simulink model "SistemaP4"  (R2023a)
settings: Solver=VariableStepAuto  StartTime=0.0  StopTime=10.0  MaxStep=1e-3  RelTol=1e-3
libraries: fl_lib x7, nesl_utility x3, slpidlib x1
settings Model: Creator=gabri  LastModifiedBy=gabri
settings DataIOCC: SaveOutput=off  SignalLogging=off  DSMLogging=off  ReturnWorkspaceOutputs=off  TimeSaveName=t
settings DebuggingCC: AlgebraicLoopMsg=none  ArtificialAlgebraicLoopMsg=none  MaxConsecutiveZCsMsg=none  ModelReferenceExtraNoncontSigs=none  OperatingPointInterfaceChecksumMismatchMsg=none

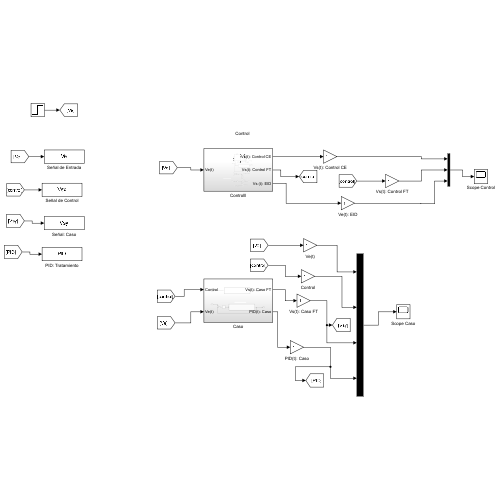
[thumbnail: Simulink's stored preview of the top-level diagram]
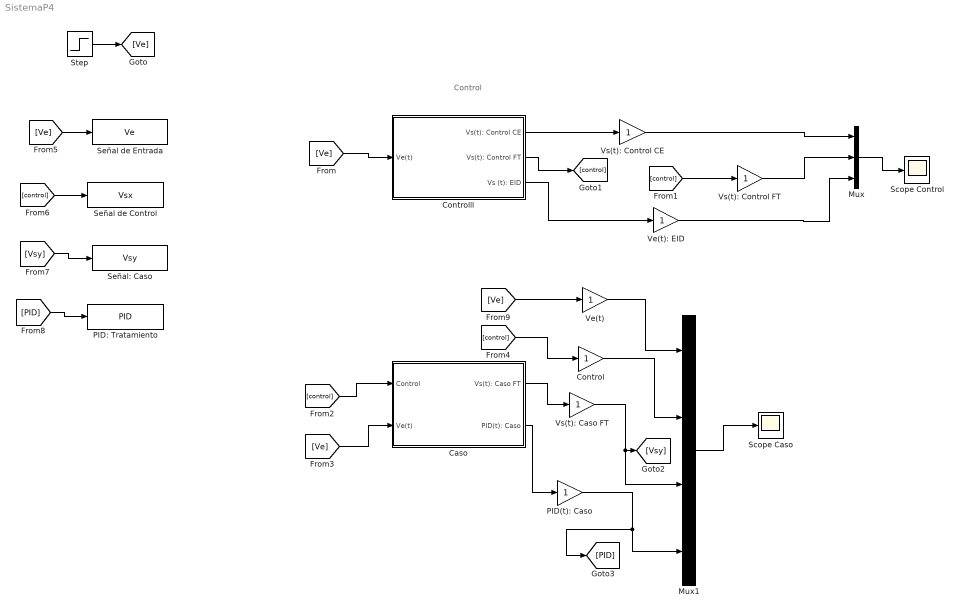
== system SistemaP4 ==
  note: Control
  Caso : Subsystem
  Control : Gain
  Controlll : Subsystem
  Mux : Mux  Inputs=3
  Mux1 : Mux
  PID(t): Caso : Gain
  PID: Tratamiento : ToWorkspace  VariableName=PID  SampleTime=-1
  Scope Caso : Scope
  Scope Control : Scope
  Señal de Control : ToWorkspace  VariableName=Vsx  SampleTime=-1
  Señal de Entrada : ToWorkspace  VariableName=Ve  SampleTime=-1
  Señal: Caso : ToWorkspace  VariableName=Vsy  SampleTime=-1
  Step : Step  Time=0  SampleTime=0
  Ve(t) : Gain
  Ve(t): EID : Gain
  Vs(t): Caso FT : Gain
  Vs(t): Control CE : Gain
  Vs(t): Control FT : Gain
  wires:
  [Ve] -> Controlll/1(Ve(t))
  Step/1 -> [Ve]
  Controlll/2(Vs(t): Control FT) -> [control]
  [control] -> Vs(t): Control FT/1
  Controlll/1(Vs(t): Control CE) -> Vs(t): Control CE/1
  Vs(t): Control CE/1 -> Mux/1
  Vs(t): Control FT/1 -> Mux/2
  Mux/1 -> Scope Control/1
  [control] -> Caso/1(Control)
  Vs(t): Caso FT/1 -> Mux1/3, [Vsy]
  Caso/2(PID(t): Caso) -> PID(t): Caso/1
  PID(t): Caso/1 -> [PID], Mux1/4
  Mux1/1 -> Scope Caso/1
  [Ve] -> Señal de Entrada/1
  [control] -> Señal de Control/1
  [Vsy] -> Señal: Caso/1
  [PID] -> PID: Tratamiento/1
  Caso/1(Vs(t): Caso FT) -> Vs(t): Caso FT/1
  [Ve] -> Caso/2(Ve(t))
  Ve(t): EID/1 -> Mux/3
  Controlll/3(Vs (t): EID) -> Ve(t): EID/1
  [Ve] -> Ve(t)/1
  Ve(t)/1 -> Mux1/1
  [control] -> Control/1
  Control/1 -> Mux1/2

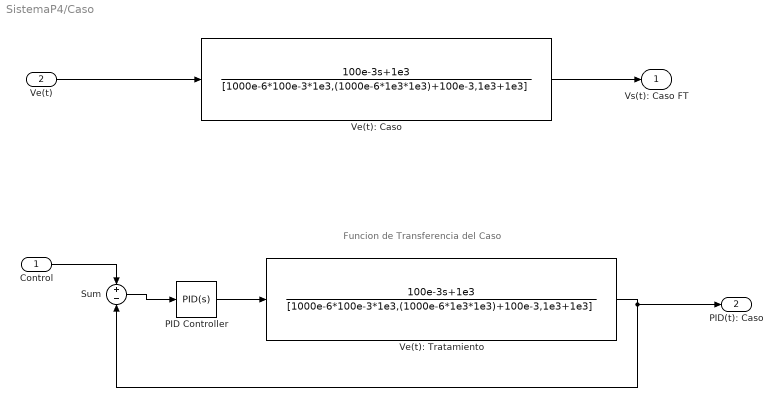
== system SistemaP4/Caso ==
  note: Funcion de Transferencia del Caso
  Control : Inport
  Ve(t) : Inport  Port=2
  PID Controller : slpidlib/PID Controller  Controller=PID  Form=Parallel  TimeDomain=Continuous-time  UseExternalTs=off  SampleTime=-1  IntegratorMethod=Forward Euler  FilterMethod=Forward Euler  ControllerParametersSource=internal  P=259.663557156946  I=12483.0782650462  UseKiTs=off  D=0.173851580929407  N=990.98480075299  UseFilter=on  TunerSelectOption=Transfer Function Based (PID Tuner App)  InitialConditionSource=internal  InitialConditionForIntegrator=0  InitialConditionForFilter=0  DifferentiatorICPrevScaledInput=0  ExternalReset=none  TrackingMode=off  Kt=1  LimitOutput=off  SatLimitsSource=internal  UpperSaturationLimit=inf  LowerSaturationLimit=-inf  LinearizeAsGain=on  AntiWindupMode=none  Kb=1  LimitIntegrator=off  UpperIntegratorSaturationLimit=inf  LowerIntegratorSaturationLimit=-inf  POutMin=[]  POutMax=[]  IOutMin=[]  IOutMax=[]  DOutMin=[]  DOutMax=[]  NOutMin=[]  NOutMax=[]  SumOutMin=[]  SumOutMax=[]  SaturationOutMin=[]  SaturationOutMax=[]  PParamMin=[]  PParamMax=[]  IParamMin=[]  IParamMax=[]  DParamMin=[]  DParamMax=[]  NParamMin=[]  NParamMax=[]  KbParamMin=[]  KbParamMax=[]  KtParamMin=[]  KtParamMax=[]  KbOutMin=[]  KbOutMax=[]  KtOutMin=[]  KtOutMax=[]  IntegratorOutMin=[]  IntegratorOutMax=[]  FilterOutMin=[]  FilterOutMax=[]  SumI1OutMin=[]  SumI1OutMax=[]  SumI2OutMin=[]  SumI2OutMax=[]  SumI3OutMin=[]  SumI3OutMax=[]  SumI4OutMin=[]  SumI4OutMax=[]  SumDOutMin=[]  SumDOutMax=[]  DifferentiatorOutMin=[]  DifferentiatorOutMax=[]  FilterDiffOutCoefMin=[]  FilterDiffOutCoefMax=[]  ReciprocalOutMin=[]  ReciprocalOutMax=[]  SumDenOutMin=[]  SumDenOutMax=[]  SumNumOutMin=[]  SumNumOutMax=[]  DivideOutMin=[]  DivideOutMax=[]  UdiffTsProdOutMin=[]  UdiffTsProdOutMax=[]  NTsProdOutMin=[]  NTsProdOutMax=[]  UintegralTsProdOutMin=[]  UintegralTsProdOutMax=[]  UngainTsProdOutMin=[]  UngainTsProdOutMax=[]  ClampingZeroOutDataTypeStr=Inherit: Inherit via back propagation  ClampingZeroOutMin=[]  ClampingZeroOutMax=[]  FilterDenConstantOutDataTypeStr=Inherit: Inherit via back propagation  FilterDenConstantOutMin=[]  FilterDenConstantOutMax=[]  PCopyOutDataTypeStr=Inherit: Inherit via back propagation  PCopyOutMin=[]  PCopyOutMax=[]  NCopyOutDataTypeStr=Inherit: Inherit via back propagation  NCopyOutMin=[]  NCopyOutMax=[]  IntegratorContinuousStateAttributes=''  IntegratorStateMustResolveToSignalObject=off  IntegratorRTWStateStorageClass=Auto  FilterContinuousStateAttributes=''  FilterStateMustResolveToSignalObject=off  FilterRTWStateStorageClass=Auto  ParallelPVariant=InternalParameters  IdealPVariant=Disabled  IVariant=InternalParameters  DVariant=InternalParameters  IntegratorVariant=Continuous  SatVariant=Disabled  AWVariant=Passthrough  PCopyVariant=Disabled  TRVariant=Disabled  FdbkBlocksVariant=Forward  IdealPFdbkVariant=Disabled  SatFdbkVariant=Disabled  DerivativeFilterVariant=ContFilter  NVariant=InternalParameters  NCopyVariant=Disabled  FilterICVariant=InternalICsFilter  IntegratorICVariant=InternalICs  ExternalResetVariant=Disabled  TRSumVariant=Passthrough  SumFdbkVariant=Disabled  SumVariant=Sum_PID  TsampFilterVariant=InternalTs  TsampNgainVariant=Passthrough  TsampIntegralVariant=Disabled_SignalSpec  ExternalSaturationOutDataTypeStr=Inherit: Same as second input
  Sum : Sum  Inputs=+-
  Ve(t): Caso : TransferFcn  Numerator=[100e-3, 1e3]  Denominator=[1000e-6*100e-3*1e3,(1000e-6*1e3*1e3)+100e-3,1e3+1e3]
  Ve(t): Tratamiento : TransferFcn  Numerator=[100e-3,1e3]  Denominator=[1000e-6*100e-3*1e3,(1000e-6*1e3*1e3)+100e-3,1e3+1e3]
  Vs(t): Caso FT : Outport
  PID(t): Caso : Outport  Port=2
  wires:
  Control/1 -> Sum/1
  Sum/1 -> PID Controller/1
  PID Controller/1 -> Ve(t): Tratamiento/1
  Ve(t): Tratamiento/1 -> Sum/2, PID(t): Caso/1
  Ve(t): Caso/1 -> Vs(t): Caso FT/1
  Ve(t)/1 -> Ve(t): Caso/1

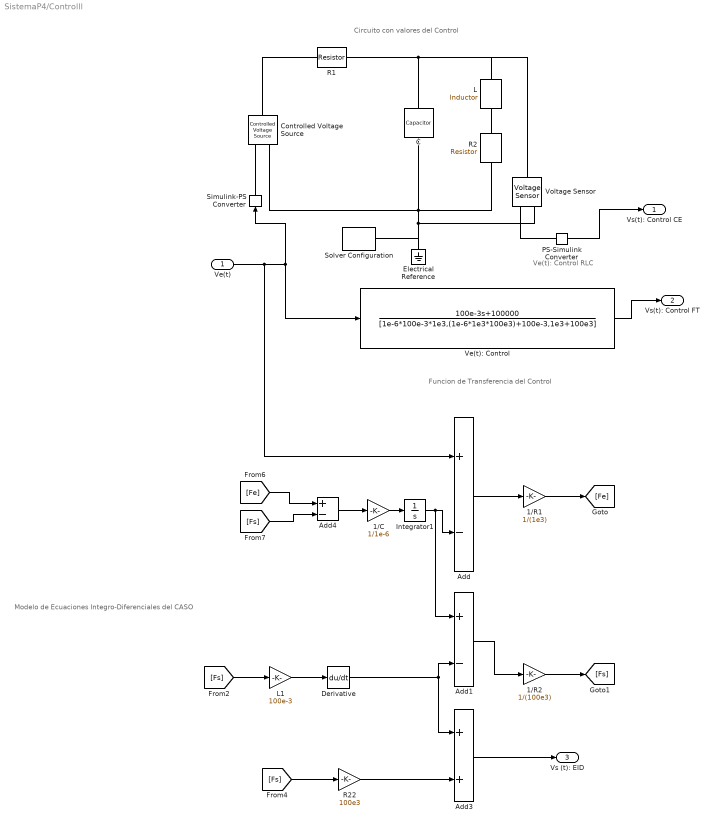
== system SistemaP4/Controlll ==
  note: Funcion de Transferencia del Control
  note: Circuito con valores del Control
  note: Ve(t): Control RLC
  note: Modelo de Ecuaciones Integro-Diferenciales del CASO
  Ve(t) : Inport
  1/C : Gain  Gain=1/1e-6
  1/R1 : Gain  Gain=1/(1e3)
  1/R2 : Gain  Gain=1/(100e3)
  Add : Sum  Inputs=+-
  Add1 : Sum  Inputs=+-
  Add3 : Sum
  Add4 : Sum  Inputs=+-
  C : fl_lib/Electrical/Electrical Elements/Capacitor  c=1e-6 F  r=1e-6 Ohm  g=0 1/Ohm  i_specify=off  i_priority=None  i=0 A  i_nominal_specify=off  i_nominal_unit=A  i_nominal_value=1  v_specify=off  v_priority=None  v=0 V  v_nominal_specify=off  v_nominal_unit=V  v_nominal_value=1  vc_specify=off  vc_priority=High  vc=0 V  vc_nominal_specify=off  vc_nominal_unit=V  vc_nominal_value=1
  Controlled Voltage Source : fl_lib/Electrical/Electrical Sources/Controlled Voltage Source
  Derivative : Derivative
  Electrical Reference : fl_lib/Electrical/Electrical Elements/Electrical Reference
  Integrator1 : Integrator
  L : fl_lib/Electrical/Electrical Elements/Inductor  l=100e-3 H  r=0 Ohm  g=1e-9 1/Ohm  i_specify=off  i_priority=None  i=0 A  i_nominal_specify=off  i_nominal_unit=A  i_nominal_value=1  v_specify=off  v_priority=None  v=0 V  v_nominal_specify=off  v_nominal_unit=V  v_nominal_value=1  i_L_specify=off  i_L_priority=High  i_L=0 A  i_L_nominal_specify=off  i_L_nominal_unit=A  i_L_nominal_value=1
  L1 : Gain  Gain=100e-3
  PS-Simulink Converter : nesl_utility/PS-Simulink Converter  PhysicalDomain=network_engine_domain  SubClassName=ps_output  LeftPortType=input  RightPortType=output  PseudoPeriodic=off  Frequencies=[]  VectorFormat=inherit  Unit=inherit  AffineConversion=off
  R1 : fl_lib/Electrical/Electrical Elements/Resistor  R=1 kOhm  i_specify=off  i_priority=None  i=0 A  i_nominal_specify=off  i_nominal_unit=A  i_nominal_value=1  v_specify=off  v_priority=None  v=0 V  v_nominal_specify=off  v_nominal_unit=V  v_nominal_value=1
  R2 : fl_lib/Electrical/Electrical Elements/Resistor  R=100 kOhm  i_specify=off  i_priority=None  i=0 A  i_nominal_specify=off  i_nominal_unit=A  i_nominal_value=1  v_specify=off  v_priority=None  v=0 V  v_nominal_specify=off  v_nominal_unit=V  v_nominal_value=1
  R22 : Gain  Gain=100e3
  Simulink-PS Converter : nesl_utility/Simulink-PS Converter  PhysicalDomain=network_engine_domain  SubClassName=ps_input  LeftPortType=input  RightPortType=output  PseudoPeriodic=off  Frequencies=[]  NoiseDistribution=none  NoiseParameters=[]  Unit=1  AffineConversion=off  FilteringAndDerivatives=provide  SimscapeFilterOrder=1  InputFilterTimeConstant=0.001  UdotUserProvided=0
  Solver Configuration : nesl_utility/Solver Configuration  PhysicalDomain=network_engine_domain  SubClassName=solver  LeftPortType=input  RightPortType=generic  Tones=[]  Harmonics=[]  SimulateNoise=off  Profile=off  UseLocalSampling=off  EnableSwitchedLinearOptims=on  FrequencyDomain=off  UseCCode=off  RelTol=0.001  AbsTol=0.001  MinStep=1e-09  ToWorkspace=off  RevertToSquareIcSolve=off  NumHomotopyIterations=100  PhasorMode=off  PhasorModeNumHarmonics=1  ConsistencySolver=NEWTON_XTOL_AFTER_FTOL  IndexReductionMethod=DerivativeReplacement  DoDC=off  ResidualTolerance=1e-09  ConsistencyTolSource=GLOBAL  ConsistencyAbsTol=0.001  ConsistencyRelTol=0.001  ConsistencyTolFactor=0.001  UseLocalSolver=off  LocalSolverChoice=NE_BACKWARD_EULER_ADVANCER  ResolveIndetEquations=on  FunctionEvalNumThread=1  LocalSolverSampleTime=0.001  DoFixedCost=off  MaxNonlinIter=3  MaxModeIter=2  ComputeImpulses=off  ImpulseIterations=2  LinearAlgebra=auto  LinearAlgebraNumThread=0  EquationFormulation=NE_TIME_EF  DelaysMemoryBudget=1024  AutomaticFiltering=on  FilteringTimeConstant=0.001  PartitionStorageMethod=AS_NEEDED  PartitionMemoryBudget=1024  PartitionMethod=ROBUST
  Ve(t): Control : TransferFcn  Numerator=[100e-3, 100000]  Denominator=[1e-6*100e-3*1e3,(1e-6*1e3*100e3)+100e-3,1e3+100e3]
  Voltage Sensor : fl_lib/Electrical/Electrical Sensors/Voltage Sensor
  Vs(t): Control CE : Outport
  Vs(t): Control FT : Outport  Port=2
  Vs (t): EID : Outport  Port=3
  wires:
  Ve(t)/1 -> Add/1, Simulink-PS Converter/1, Ve(t): Control/1
  PS-Simulink Converter/1 -> Vs(t): Control CE/1
  Ve(t): Control/1 -> Vs(t): Control FT/1
  Add3/1 -> Vs (t): EID/1
  Add1/1 -> 1/R2/1
  1/R2/1 -> [Fs]
  [Fs] -> R22/1
  R22/1 -> Add3/2
  [Fs] -> L1/1
  L1/1 -> Derivative/1
  Derivative/1 -> Add3/1, Add1/2
  [Fe] -> Add4/1
  Integrator1/1 -> Add1/1, Add/2
  1/C/1 -> Integrator1/1
  Add4/1 -> 1/C/1
  Add/1 -> 1/R1/1
  [Fs] -> Add4/2
  1/R1/1 -> [Fe]
  connections:
  Simulink-PS Converter/RConn1 -- Controlled Voltage Source/RConn1
  Controlled Voltage Source/RConn2 -- R2/RConn1 -- Solver Configuration/RConn1 -- Electrical Reference/LConn1 -- Voltage Sensor/RConn2 -- C/RConn1
  Voltage Sensor/RConn1 -- PS-Simulink Converter/LConn1
  Controlled Voltage Source/LConn1 -- R1/LConn1
  R1/RConn1 -- Voltage Sensor/LConn1 -- L/LConn1 -- C/LConn1
  L/RConn1 -- R2/LConn1
